simulink model "Signed_Rate_Limiter"  (R2023b)
settings: Solver=VariableStepAuto  StartTime=0.0  StopTime=3  FixedStep=.02  MaxStep=.02  RelTol=1e-3
libraries: fl_lib x3, nesl_utility x2, simulink x1, Simulation_lib x1, Controls_Components_lib x1
settings Model: Creator=FIRSTMentor  LastModifiedBy=ander
settings OptimizationCC: BlockReduction=off  DefaultParameterBehavior=Inlined  BufferReuse=off

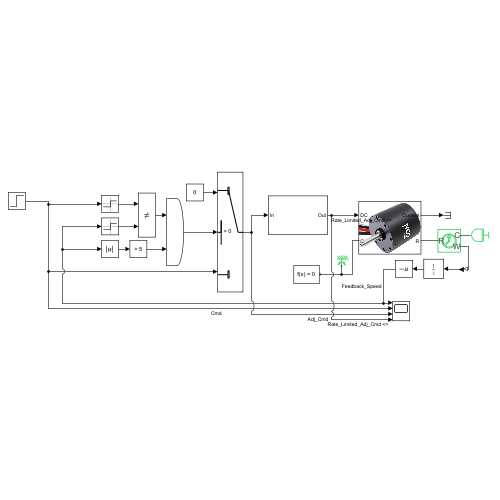
[thumbnail: Simulink's stored preview of the top-level diagram]
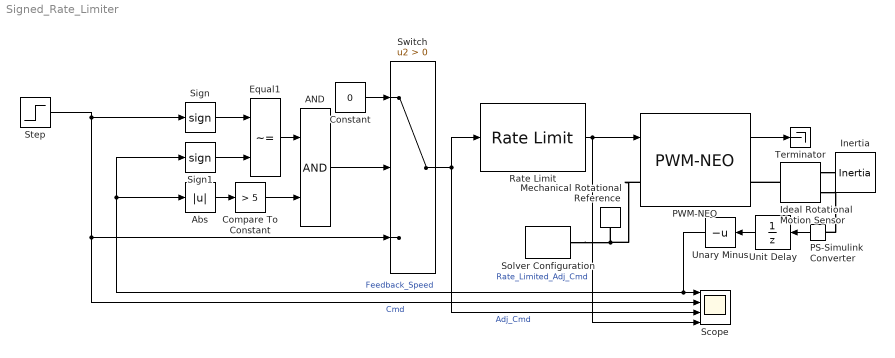
== system Signed_Rate_Limiter ==
  AND : Logic  IconShape=distinctive  AllPortsSameDT=off  OutDataTypeStr=boolean
  Abs : Abs  SaturateOnIntegerOverflow=off
  Compare To Constant : simulink/Logic and Bit Operations/Compare To Constant  relop=>  const=5  OutDataTypeStr=boolean
  Constant : Constant  Value=0
  Equal1 : RelationalOperator  Operator=~=  OutDataTypeStr=boolean  RndMeth=Simplest  InputSameDT=off
  Ideal Rotational Motion Sensor : fl_lib/Mechanical/Mechanical Sensors/Ideal Rotational Motion Sensor  reference=foundation.enum.MeasurementReference.difference  acceleration_port=false  velocity_port=true  position_port=false  wrap_angle=false  offset=0 rad
      settings: InternalSimscapePortConfiguration="{\"Bottom\":[],\"Left\":[{\"id\":\"R\",\"label\":\"R\",\"type\":\"foundation.mechanical.rotational.rotational\"}],\"Right\":[{\"id\":\"C\",\"label\":\"C\",\"type\":\"foundation.mechanical.rotational.rotational\"},{\"id\":\"W\",\"label\":\"W\",\"type\":\"output\"}],\"Top\":[]}"
  Inertia : fl_lib/Mechanical/Rotational Elements/Inertia  inertia=.5 lbm*in^2  num_ports=foundation.enum.numPorts2.one  w_specify=off  w_priority=High  w=0 rad/s  w_nominal_specify=off  w_nominal_unit=rad/s  w_nominal_value=1  t_specify=off  t_priority=None  t=0 N*m  t_nominal_specify=off  t_nominal_unit=N*m  t_nominal_value=1
  Mechanical Rotational Reference : fl_lib/Mechanical/Rotational Elements/Mechanical Rotational Reference
  PS-Simulink Converter : nesl_utility/PS-Simulink Converter  PhysicalDomain=network_engine_domain  SubClassName=ps_output  LeftPortType=input  RightPortType=output  PseudoPeriodic=off  Frequencies=[]  VectorFormat=inherit  Unit=inherit  AffineConversion=off
  PWM-NEO : Simulation_lib/PWM-NEO  SystemSampleTime=-1  VariantActivationTime=update diagram  AllowFlexibleInterface=on  Latency=0  AutoFrameSizeCalculation=off
  Rate Limit : Controls_Components_lib/Rate Limit  Rate_Limit_Inc=1/0.75*0.02  Rate_Limit_Dec=-1/0.25*0.02  Approaching_Zero_Error_Threshold=0.2  Approaching_Zero_Final_Scale_Factor=0.01  Approaching_NonZero_Error_Threshold=0.2  Approaching_NonZero_Final_Scale_Factor=0.1
  Scope : Scope  NumInputPorts=4
  Sign : Signum
  Sign1 : Signum
  Solver Configuration : nesl_utility/Solver Configuration  PhysicalDomain=network_engine_domain  SubClassName=solver  LeftPortType=input  RightPortType=generic  Tones=[]  Harmonics=[]  SimulateNoise=off  Profile=off  UseLocalSampling=off  EnableSwitchedLinearOptims=on  FrequencyDomain=off  UseCCode=off  RelTol=0.001  AbsTol=0.001  MinStep=1e-09  ToWorkspace=off  RevertToSquareIcSolve=off  NumHomotopyIterations=100  PhasorMode=off  PhasorModeNumHarmonics=1  ConsistencySolver=NEWTON_XTOL_AFTER_FTOL  IndexReductionMethod=DerivativeReplacement  DoDC=off  ResidualTolerance=1e-09  ConsistencyTolSource=GLOBAL  ConsistencyAbsTol=0.001  ConsistencyRelTol=0.001  ConsistencyTolFactor=0.001  UseLocalSolver=off  LocalSolverChoice=NE_BACKWARD_EULER_ADVANCER  ResolveIndetEquations=on  FunctionEvalNumThread=1  LocalSolverSampleTime=0.001  DoFixedCost=off  MaxNonlinIter=3  MaxModeIter=2  ComputeImpulses=off  ImpulseIterations=2  LinearAlgebra=auto  LinearAlgebraNumThread=0  EquationFormulation=NE_TIME_EF  DelaysMemoryBudget=1024  AutomaticFiltering=on  FilteringTimeConstant=0.001  PartitionStorageMethod=AS_NEEDED  PartitionMemoryBudget=1024  PartitionMethod=ROBUST  MultibodyUseLocalSolver=off  MultibodyLocalSolverChoice=ODE1  MultibodyLocalSolverSampleTime=0.001
  Step : Step  Before=-1  SampleTime=0
  Switch : Switch  Criteria=u2 > Threshold  SaturateOnIntegerOverflow=off  InputSameDT=off
  Terminator : Terminator
  Unary Minus : UnaryMinus
  Unit Delay : UnitDelay  SampleTime=-1  HasFrameUpgradeWarning=on
  wires:
  PWM-NEO/1 -> Terminator/1
  PS-Simulink Converter/1 -> Unit Delay/1
  Step/1 -> Scope/2, Switch/3, Sign/1  "Cmd"
  Constant/1 -> Switch/1
  Switch/1 -> Rate Limit/1, Scope/3  "Adj_Cmd"
  Rate Limit/1 -> PWM-NEO/1, Scope/4  "Rate_Limited_Adj_Cmd"
  Sign/1 -> Equal1/1
  Sign1/1 -> Equal1/2
  Equal1/1 -> AND/1
  AND/1 -> Switch/2
  Abs/1 -> Compare To Constant/1
  Unit Delay/1 -> Unary Minus/1
  Unary Minus/1 -> Sign1/1, Abs/1, Scope/1  "Feedback_Speed"
  Compare To Constant/1 -> AND/2
  connections:
  PWM-NEO/LConn1 -- Solver Configuration/RConn1 -- Mechanical Rotational Reference/LConn1
  Ideal Rotational Motion Sensor/LConn1 -- PWM-NEO/RConn1
  Ideal Rotational Motion Sensor/RConn1 -- Inertia/LConn1
  Ideal Rotational Motion Sensor/RConn2 -- PS-Simulink Converter/LConn1
